simulink model "TurnLight1"  (R2020b)
settings: Solver=FixedStepDiscrete  StartTime=0.0  StopTime=10.0  FixedStep=0.01  RelTol=1e-3
values from neighbouring files (symbols this model uses):
  EBL_NO_REQ = 0    [TurnLightUserdata.m]
  EBL_REQ = 1    [TurnLightUserdata.m]
  HAZARDQR_OFF = 0    [TurnLightUserdata.m]
  HAZARDQR_ON = 1    [TurnLightUserdata.m]
  HAZARDRQ_OFF = 0    [TurnLightUserdata.m]
  HAZARDRQ_ON = 1    [TurnLightUserdata.m]
  HAZARDSW_OFF = 0    [TurnLightUserdata.m]
  HAZARDSW_ON = 1    [TurnLightUserdata.m]
  IGN_ACC = 1    [TurnLightUserdata.m]
  IGN_IGNST = 3    [TurnLightUserdata.m]
  IGN_OFF = 0    [TurnLightUserdata.m]
  IGN_ON = 2    [TurnLightUserdata.m]
  NO_CRASH = 0    [TurnLightUserdata.m]
  TLCC_ON = 1    [TurnLightUserdata.m]
  TLFB_OFF = 0    [TurnLightUserdata.m]
  TLFB_OPEN = 2    [TurnLightUserdata.m]
  TLFB_SHORT = 1    [TurnLightUserdata.m]
  TLSR_LEFT_ON = 1    [TurnLightUserdata.m]
  TLSR_OFF = 0    [TurnLightUserdata.m]
  TLSR_RIGHT_ON = 2    [TurnLightUserdata.m]
  TLSW_LEFT = 1    [TurnLightUserdata.m]
  TLSW_OFF = 0    [TurnLightUserdata.m]
  TLSW_RIGHT = 2    [TurnLightUserdata.m]
  TLSWMODE_FLASH0 = 0    [TurnLightUserdata.m]
  TLSWMODE_FLASH3 = 1    [TurnLightUserdata.m]
  TLSWMODE_FLASHLONG = 2    [TurnLightUserdata.m]
  VS_VALID = 1    [TurnLightUserdata.m]
undefined symbols (not defined in the file or in its folder): ComplexTurnLightONOFFType, ComplexTurnLightPositionType, TurnLightCtrlPara, TurnLightService_TurnLightControl_Operation
settings Model: Creator=Wangjianwen  LastModifiedBy=Wangjianwen
settings DataIOCC: SaveFormat=StructureWithTime
settings OptimizationCC: DefaultParameterBehavior=Inlined  EnhancedBackFolding=on  PassReuseOutputArgsAs=Individual arguments  ZeroExternalMemoryAtStartup=off  ZeroInternalMemoryAtStartup=off  OptimizeBlockOrder=speed  DifferentSizesBufferReuse=on  OptimizationCustomize=off  EfficientTunableParamExpr=on
settings DebuggingCC: ParameterTunabilityLossMsg=error  SFUnusedDataAndEventsDiag=none
settings HardwareCC: ProdLongLongMode=on
settings ModelReferenceCC: ModelReferenceNumInstancesAllowed=Single
settings SFSimCC: MATLABDynamicMemAlloc=off
settings RTWCC: Description=AUTOSAR  SystemTargetFile=autosar.tlc  GenCodeOnly=on  TemplateMakefile=ert_default_tmf
settings CodeAppCC: ForceParamTrailComments=on  IgnoreCustomStorageClasses=off  OperatorAnnotations=on  SimulinkDataObjDesc=on  SFDataObjDesc=on  InsertBlockDesc=on
settings STFCustomTargetCC: TargetLangStandard=C99 (ISO)  MultiwordLength=256  ParMdlRefBuildCompliant=on  CompOptLevelCompliant=on  ConcurrentExecutionCompliant=off  IncludeMdlTerminateFcn=off  CombineOutputUpdateFcns=on  SuppressErrorStatus=on  ERTCustomFileBanners=on  SupportNonFinite=off  SupportComplex=off  SupportContinuousTime=off  SupportNonInlinedSFcns=off  RemoveResetFunc=on  MATLABClassNameForMDSCustomization=Simulink.SoftwareTarget.ERTCustomization  CPPClassGenCompliant=off  AutosarCompliant=on  GRTInterface=off  UseToolchainInfoCompliant=on  LookupTableObjectStructAxisOrder=2,1,3,4,...  LUTObjectStructOrderEvenSpacing=Size,Table,Breakpoints  SystemTargetFile=autosar.tlc
settings ERTTargetCC: TargetLangStandard=C99 (ISO)  ConcurrentExecutionCompliant=off  IncludeMdlTerminateFcn=off  SuppressErrorStatus=on  SupportNonFinite=off  SupportComplex=off  ModelStepFunctionPrototypeControlCompliant=off  CPPClassGenCompliant=off  AutosarCompliant=on  LookupTableObjectStructAxisOrder=2,1,3,4,...  LUTObjectStructOrderEvenSpacing=Size,Table,Breakpoints  InlinedParameterPlacement=NonHierarchical  ERTCustomFileTemplate=example_file_process.tlc

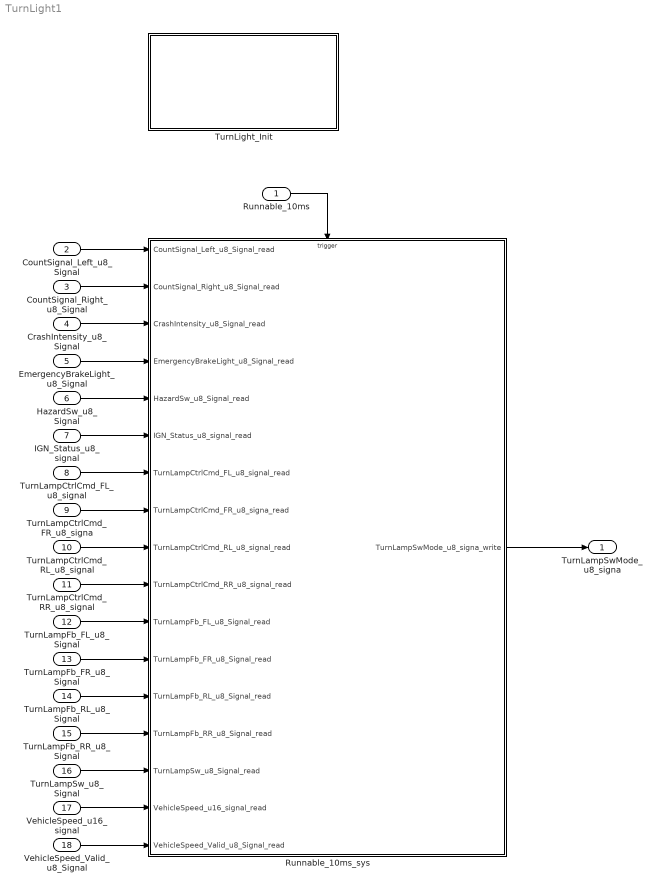
== system TurnLight1 ==
  Runnable_10ms : Inport  SampleTime=0.01  OutputFunctionCall=on
  CountSignal_Left_u8_Signal : Inport  Port=2  OutDataTypeStr=uint8  PortDimensions=1
  CountSignal_Right_u8_Signal : Inport  Port=3  OutDataTypeStr=uint8  PortDimensions=1
  CrashIntensity_u8_Signal : Inport  Port=4  OutDataTypeStr=uint8  PortDimensions=1
  EmergencyBrakeLight_u8_Signal : Inport  Port=5  OutDataTypeStr=uint8  PortDimensions=1
  HazardSw_u8_Signal : Inport  Port=6  OutDataTypeStr=uint8  PortDimensions=1
  IGN_Status_u8_signal : Inport  Port=7  OutDataTypeStr=uint8  PortDimensions=1
  TurnLampCtrlCmd_FL_u8_signal : Inport  Port=8  OutDataTypeStr=uint8  PortDimensions=1
  TurnLampCtrlCmd_FR_u8_signa : Inport  Port=9  OutDataTypeStr=uint8  PortDimensions=1
  TurnLampCtrlCmd_RL_u8_signal : Inport  Port=10  OutDataTypeStr=uint8  PortDimensions=1
  TurnLampCtrlCmd_RR_u8_signal : Inport  Port=11  OutDataTypeStr=uint64  PortDimensions=1
  TurnLampFb_FL_u8_Signal : Inport  Port=12  OutDataTypeStr=uint8  PortDimensions=1
  TurnLampFb_FR_u8_Signal : Inport  Port=13  OutDataTypeStr=uint8  PortDimensions=1
  TurnLampFb_RL_u8_Signal : Inport  Port=14  OutDataTypeStr=uint8  PortDimensions=1
  TurnLampFb_RR_u8_Signal : Inport  Port=15  OutDataTypeStr=uint8  PortDimensions=1
  TurnLampSw_u8_Signal : Inport  Port=16  OutDataTypeStr=uint8  PortDimensions=1
  VehicleSpeed_u16_signal : Inport  Port=17  OutDataTypeStr=uint16  PortDimensions=1
  VehicleSpeed_Valid_u8_Signal : Inport  Port=18  OutDataTypeStr=uint8  PortDimensions=1
  Runnable_10ms_sys : Subsystem
  TurnLight_Init : Subsystem
  TurnLampSwMode_u8_signa : Outport  OutDataTypeStr=uint8  PortDimensions=1
  wires:
  CountSignal_Left_u8_Signal/1 -> Runnable_10ms_sys/1(CountSignal_Left_u8_Signal_read)
  CountSignal_Right_u8_Signal/1 -> Runnable_10ms_sys/2(CountSignal_Right_u8_Signal_read)
  CrashIntensity_u8_Signal/1 -> Runnable_10ms_sys/3(CrashIntensity_u8_Signal_read)
  EmergencyBrakeLight_u8_Signal/1 -> Runnable_10ms_sys/4(EmergencyBrakeLight_u8_Signal_read)
  HazardSw_u8_Signal/1 -> Runnable_10ms_sys/5(HazardSw_u8_Signal_read)
  IGN_Status_u8_signal/1 -> Runnable_10ms_sys/6(IGN_Status_u8_signal_read)
  TurnLampCtrlCmd_FL_u8_signal/1 -> Runnable_10ms_sys/7(TurnLampCtrlCmd_FL_u8_signal_read)
  TurnLampCtrlCmd_FR_u8_signa/1 -> Runnable_10ms_sys/8(TurnLampCtrlCmd_FR_u8_signa_read)
  TurnLampCtrlCmd_RL_u8_signal/1 -> Runnable_10ms_sys/9(TurnLampCtrlCmd_RL_u8_signal_read)
  TurnLampCtrlCmd_RR_u8_signal/1 -> Runnable_10ms_sys/10(TurnLampCtrlCmd_RR_u8_signal_read)
  TurnLampFb_FL_u8_Signal/1 -> Runnable_10ms_sys/11(TurnLampFb_FL_u8_Signal_read)
  TurnLampFb_FR_u8_Signal/1 -> Runnable_10ms_sys/12(TurnLampFb_FR_u8_Signal_read)
  TurnLampFb_RL_u8_Signal/1 -> Runnable_10ms_sys/13(TurnLampFb_RL_u8_Signal_read)
  TurnLampFb_RR_u8_Signal/1 -> Runnable_10ms_sys/14(TurnLampFb_RR_u8_Signal_read)
  TurnLampSw_u8_Signal/1 -> Runnable_10ms_sys/15(TurnLampSw_u8_Signal_read)
  VehicleSpeed_u16_signal/1 -> Runnable_10ms_sys/16(VehicleSpeed_u16_signal_read)
  VehicleSpeed_Valid_u8_Signal/1 -> Runnable_10ms_sys/17(VehicleSpeed_Valid_u8_Signal_read)
  Runnable_10ms_sys/1(TurnLampSwMode_u8_signa_write) -> TurnLampSwMode_u8_signa/1
  Runnable_10ms/1 -> Runnable_10ms_sys/Trigger

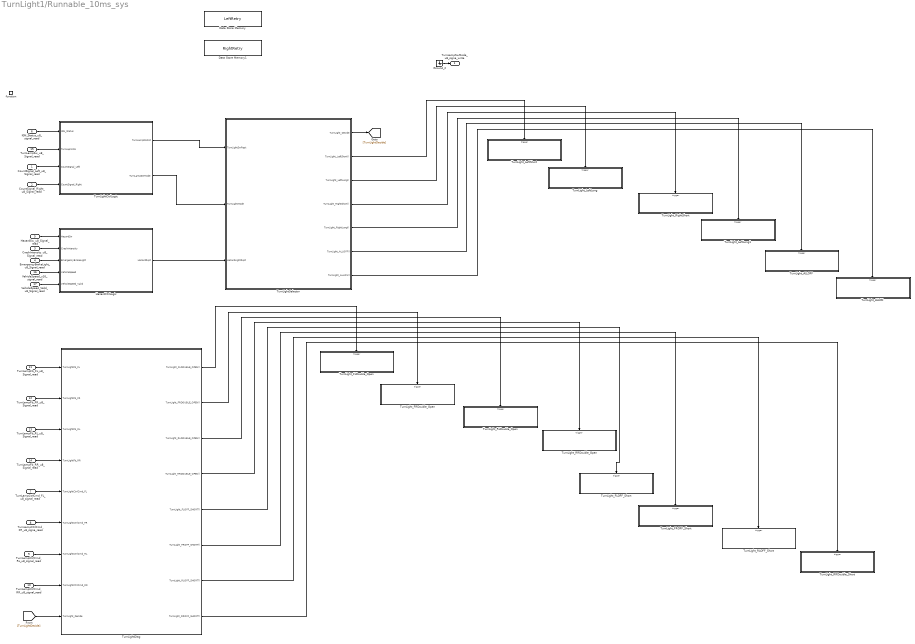
== system TurnLight1/Runnable_10ms_sys ==
  CountSignal_Left_u8_Signal_read : Inport
  CountSignal_Right_u8_Signal_read : Inport  Port=2
  CrashIntensity_u8_Signal_read : Inport  Port=3
  EmergencyBrakeLight_u8_Signal_read : Inport  Port=4
  HazardSw_u8_Signal_read : Inport  Port=5
  IGN_Status_u8_signal_read : Inport  Port=6
  TurnLampCtrlCmd_FL_u8_signal_read : Inport  Port=7
  TurnLampCtrlCmd_FR_u8_signa_read : Inport  Port=8
  TurnLampCtrlCmd_RL_u8_signal_read : Inport  Port=9
  TurnLampCtrlCmd_RR_u8_signal_read : Inport  Port=10
  TurnLampFb_FL_u8_Signal_read : Inport  Port=11
  TurnLampFb_FR_u8_Signal_read : Inport  Port=12
  TurnLampFb_RL_u8_Signal_read : Inport  Port=13
  TurnLampFb_RR_u8_Signal_read : Inport  Port=14
  TurnLampSw_u8_Signal_read : Inport  Port=15
  VehicleSpeed_u16_signal_read : Inport  Port=16
  VehicleSpeed_Valid_u8_Signal_read : Inport  Port=17
  function : TriggerPort  TriggerType=function-call  VariantControl=(inherit)  SampleTimeType=periodic  SampleTime=-1
  Data Store Memory : DataStoreMemory  DataStoreName=LeftRetry  ReadBeforeWriteMsg=warning  WriteAfterWriteMsg=warning  WriteAfterReadMsg=warning  ShowAdditionalParam=off  OutDataTypeStr=uint8
  Data Store Memory1 : DataStoreMemory  DataStoreName=RightRetry  ReadBeforeWriteMsg=warning  WriteAfterWriteMsg=warning  WriteAfterReadMsg=warning  ShowAdditionalParam=off  OutDataTypeStr=uint8
  Ground_2 : Ground
  HazardCtrlLogic : Stateflow chart  TreatAsAtomicUnit=on
  TurnLightCtrlLogic : Stateflow chart  TreatAsAtomicUnit=on
  TurnLightDiag : Stateflow chart  TreatAsAtomicUnit=on
  TurnLightSelector : Stateflow chart  TreatAsAtomicUnit=on
  TurnLight_ALLOFF : Subsystem
  TurnLight_ALLON : Subsystem
  TurnLight_FLDouble_Open : Subsystem
  TurnLight_FLOFF_Short : Subsystem
  TurnLight_FRDouble_Open : Subsystem
  TurnLight_FROFF_Short : Subsystem
  TurnLight_LeftLong : Subsystem
  TurnLight_LeftLong1 : Subsystem
  TurnLight_LeftShort : Subsystem
  TurnLight_RLDouble_Open : Subsystem
  TurnLight_RLOFF_Short : Subsystem
  TurnLight_RRDouble_Open : Subsystem
  TurnLight_RRDouble_Short : Subsystem
  TurnLight_RightShort : Subsystem
  TurnLampSwMode_u8_signa_write : Outport
      settings: EnsureOutportIsVirtual=on
  wires:
  CountSignal_Left_u8_Signal_read/1 -> TurnLightCtrlLogic/3(CountSignal_Left)
  CountSignal_Right_u8_Signal_read/1 -> TurnLightCtrlLogic/4(CountSignal_Right)
  CrashIntensity_u8_Signal_read/1 -> HazardCtrlLogic/2(CrashIntensity)
  EmergencyBrakeLight_u8_Signal_read/1 -> HazardCtrlLogic/3(EmergencyBrakeLight)
  HazardSw_u8_Signal_read/1 -> HazardCtrlLogic/1(HazardSw)
  TurnLampCtrlCmd_FL_u8_signal_read/1 -> TurnLightDiag/5(TurnLightCtrlCmd_FL)
  TurnLampCtrlCmd_FR_u8_signa_read/1 -> TurnLightDiag/6(TurnLightCtrlCmd_FR)
  TurnLampCtrlCmd_RL_u8_signal_read/1 -> TurnLightDiag/7(TurnLightCtrlCmd_RL)
  TurnLampCtrlCmd_RR_u8_signal_read/1 -> TurnLightDiag/8(TurnLightCtrlCmd_RR)
  TurnLampFb_FL_u8_Signal_read/1 -> TurnLightDiag/1(TurnLightFb_FL)
  TurnLampFb_FR_u8_Signal_read/1 -> TurnLightDiag/2(TurnLightFb_FR)
  TurnLampFb_RL_u8_Signal_read/1 -> TurnLightDiag/3(TurnLightFb_RL)
  TurnLampFb_RR_u8_Signal_read/1 -> TurnLightDiag/4(TurnLightFb_RR)
  TurnLampSw_u8_Signal_read/1 -> TurnLightCtrlLogic/2(TurnLapmSW)
  VehicleSpeed_u16_signal_read/1 -> HazardCtrlLogic/4(VehicleSpeed)
  VehicleSpeed_Valid_u8_Signal_read/1 -> HazardCtrlLogic/5(VehicleSpeed_Valid)
  Ground_2/1 -> TurnLampSwMode_u8_signa_write/1
  IGN_Status_u8_signal_read/1 -> TurnLightCtrlLogic/1(IGN_Status)
  TurnLightCtrlLogic/1(TurnLampSWRst) -> TurnLightSelector/1(TurnLightSwRqst)
  HazardCtrlLogic/1(HazardRqst) -> TurnLightSelector/3(HazardLightRqst)
  TurnLightCtrlLogic/2(TurnLampSWMode) -> TurnLightSelector/2(TurnLightMode)
  TurnLightSelector/2(TurnLight_LeftShort()) -> TurnLight_LeftShort/Trigger
  TurnLightSelector/3(TurnLight_LeftLong()) -> TurnLight_LeftLong/Trigger
  TurnLightSelector/4(TurnLight_RightShort()) -> TurnLight_RightShort/Trigger
  TurnLightSelector/5(TurnLight_RightLong()) -> TurnLight_LeftLong1/Trigger
  TurnLightSelector/6(TurnLight_ALLOFF()) -> TurnLight_ALLOFF/Trigger
  TurnLightSelector/7(TurnLight_ALLON()) -> TurnLight_ALLON/Trigger
  TurnLightSelector/1(TurnLight_Decide) -> [TurnLightDecide]
  [TurnLightDecide] -> TurnLightDiag/9(TurnLight_Decide)
  TurnLightDiag/1(TurnLight_FLDOUBLE_OPEN()) -> TurnLight_FLDouble_Open/Trigger
  TurnLightDiag/2(TurnLight_FRDOUBLE_OPEN()) -> TurnLight_FRDouble_Open/Trigger
  TurnLightDiag/3(TurnLight_RLDOUBLE_OPEN()) -> TurnLight_RLDouble_Open/Trigger
  TurnLightDiag/4(TurnLight_RRDOUBLE_OPEN()) -> TurnLight_RRDouble_Open/Trigger
  TurnLightDiag/5(TurnLight_FLOFF_SHORT()) -> TurnLight_FLOFF_Short/Trigger
  TurnLightDiag/6(TurnLight_FROFF_SHORT()) -> TurnLight_FROFF_Short/Trigger
  TurnLightDiag/7(TurnLight_RLOFF_SHORT()) -> TurnLight_RLOFF_Short/Trigger
  TurnLightDiag/8(TurnLight_RROFF_SHORT()) -> TurnLight_RRDouble_Short/Trigger

== system TurnLight1/TurnLight_Init ==
  Event Listener : EventListener  EventName=reset

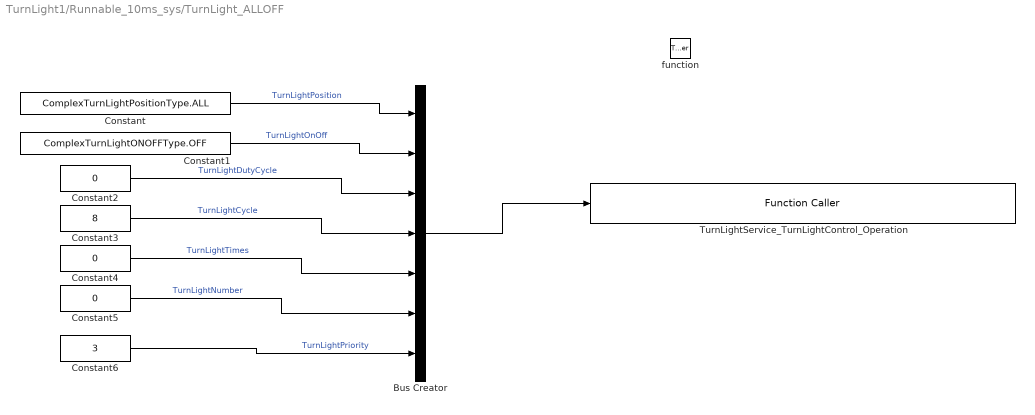
== system TurnLight1/Runnable_10ms_sys/TurnLight_ALLOFF ==
  function : TriggerPort  TriggerType=function-call  VariantControl=Variant
  Bus Creator : BusCreator  Inputs=7  OutDataTypeStr=Bus: TurnLightService  NonVirtualBus=on
  Constant : Constant  Value=ComplexTurnLightPositionType.ALL  OutDataTypeStr=Enum: ComplexTurnLightPositionType
  Constant1 : Constant  Value=ComplexTurnLightONOFFType.OFF  OutDataTypeStr=Enum: ComplexTurnLightONOFFType
  Constant2 : Constant  Value=0  OutDataTypeStr=uint8
  Constant3 : Constant  Value=8  OutDataTypeStr=uint8
  Constant4 : Constant  Value=0  OutDataTypeStr=uint8
  Constant5 : Constant  Value=0  OutDataTypeStr=uint8
  Constant6 : Constant  Value=3  OutDataTypeStr=uint8
  TurnLightService_TurnLightControl_Operation : FunctionCaller  FunctionPrototype=TurnLightService_TurnLightControl_Operation(TurnLightCtrlPara)  InputArgumentSpecifications=P_TurnLightService
  wires:
  Constant6/1 -> Bus Creator/7  "TurnLightPriority"
  Constant5/1 -> Bus Creator/6  "TurnLightNumber"
  Constant4/1 -> Bus Creator/5  "TurnLightTimes"
  Constant3/1 -> Bus Creator/4  "TurnLightCycle"
  Constant2/1 -> Bus Creator/3  "TurnLightDutyCycle"
  Constant1/1 -> Bus Creator/2  "TurnLightOnOff"
  Constant/1 -> Bus Creator/1  "TurnLightPosition"
  Bus Creator/1 -> TurnLightService_TurnLightControl_Operation/1

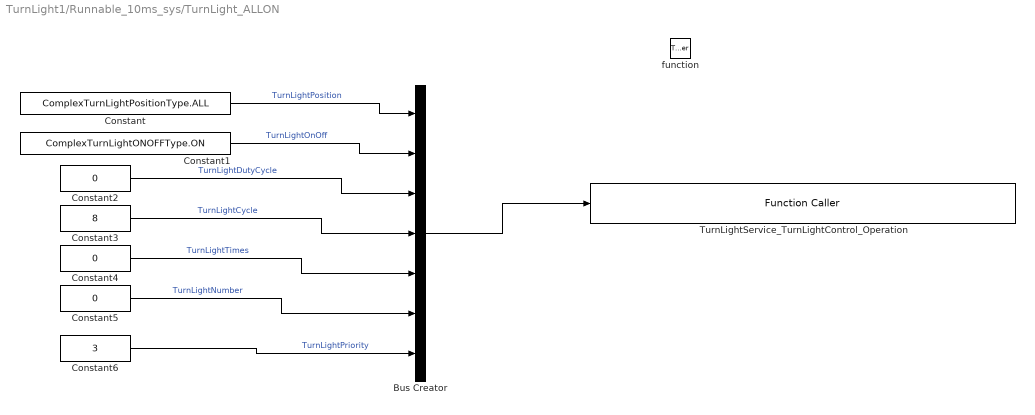
== system TurnLight1/Runnable_10ms_sys/TurnLight_ALLON ==
  function : TriggerPort  TriggerType=function-call  VariantControl=Variant
  Bus Creator : BusCreator  Inputs=7  OutDataTypeStr=Bus: TurnLightService  NonVirtualBus=on
  Constant : Constant  Value=ComplexTurnLightPositionType.ALL  OutDataTypeStr=Enum: ComplexTurnLightPositionType
  Constant1 : Constant  Value=ComplexTurnLightONOFFType.ON  OutDataTypeStr=Enum: ComplexTurnLightONOFFType
  Constant2 : Constant  Value=0  OutDataTypeStr=uint8
  Constant3 : Constant  Value=8  OutDataTypeStr=uint8
  Constant4 : Constant  Value=0  OutDataTypeStr=uint8
  Constant5 : Constant  Value=0  OutDataTypeStr=uint8
  Constant6 : Constant  Value=3  OutDataTypeStr=uint8
  TurnLightService_TurnLightControl_Operation : FunctionCaller  FunctionPrototype=TurnLightService_TurnLightControl_Operation(TurnLightCtrlPara)  InputArgumentSpecifications=P_TurnLightService
  wires:
  Bus Creator/1 -> TurnLightService_TurnLightControl_Operation/1
  Constant/1 -> Bus Creator/1  "TurnLightPosition"
  Constant1/1 -> Bus Creator/2  "TurnLightOnOff"
  Constant2/1 -> Bus Creator/3  "TurnLightDutyCycle"
  Constant3/1 -> Bus Creator/4  "TurnLightCycle"
  Constant4/1 -> Bus Creator/5  "TurnLightTimes"
  Constant5/1 -> Bus Creator/6  "TurnLightNumber"
  Constant6/1 -> Bus Creator/7  "TurnLightPriority"

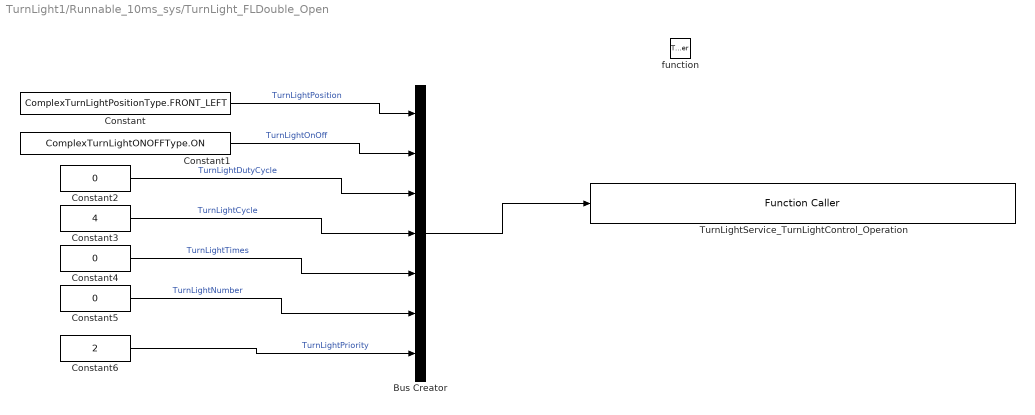
== system TurnLight1/Runnable_10ms_sys/TurnLight_FLDouble_Open ==
  function : TriggerPort  TriggerType=function-call  VariantControl=Variant
  Bus Creator : BusCreator  Inputs=7  OutDataTypeStr=Bus: TurnLightService  NonVirtualBus=on
  Constant : Constant  Value=ComplexTurnLightPositionType.FRONT_LEFT  OutDataTypeStr=Enum: ComplexTurnLightPositionType
  Constant1 : Constant  Value=ComplexTurnLightONOFFType.ON  OutDataTypeStr=Enum: ComplexTurnLightONOFFType
  Constant2 : Constant  Value=0  OutDataTypeStr=uint8
  Constant3 : Constant  Value=4  OutDataTypeStr=uint8
  Constant4 : Constant  Value=0  OutDataTypeStr=uint8
  Constant5 : Constant  Value=0  OutDataTypeStr=uint8
  Constant6 : Constant  Value=2  OutDataTypeStr=uint8
  TurnLightService_TurnLightControl_Operation : FunctionCaller  FunctionPrototype=TurnLightService_TurnLightControl_Operation(TurnLightCtrlPara)  InputArgumentSpecifications=P_TurnLightService
  wires:
  Bus Creator/1 -> TurnLightService_TurnLightControl_Operation/1
  Constant/1 -> Bus Creator/1  "TurnLightPosition"
  Constant1/1 -> Bus Creator/2  "TurnLightOnOff"
  Constant2/1 -> Bus Creator/3  "TurnLightDutyCycle"
  Constant3/1 -> Bus Creator/4  "TurnLightCycle"
  Constant4/1 -> Bus Creator/5  "TurnLightTimes"
  Constant5/1 -> Bus Creator/6  "TurnLightNumber"
  Constant6/1 -> Bus Creator/7  "TurnLightPriority"

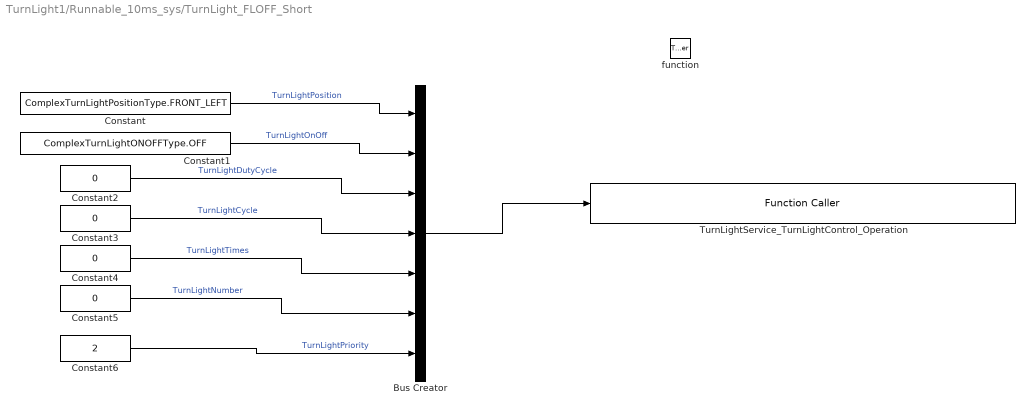
== system TurnLight1/Runnable_10ms_sys/TurnLight_FLOFF_Short ==
  function : TriggerPort  TriggerType=function-call  VariantControl=Variant
  Bus Creator : BusCreator  Inputs=7  OutDataTypeStr=Bus: TurnLightService  NonVirtualBus=on
  Constant : Constant  Value=ComplexTurnLightPositionType.FRONT_LEFT  OutDataTypeStr=Enum: ComplexTurnLightPositionType
  Constant1 : Constant  Value=ComplexTurnLightONOFFType.OFF  OutDataTypeStr=Enum: ComplexTurnLightONOFFType
  Constant{2..5} (4 alike) : Constant  Value=0  OutDataTypeStr=uint8
  Constant6 : Constant  Value=2  OutDataTypeStr=uint8
  TurnLightService_TurnLightControl_Operation : FunctionCaller  FunctionPrototype=TurnLightService_TurnLightControl_Operation(TurnLightCtrlPara)  InputArgumentSpecifications=P_TurnLightService
  wires:
  Constant6/1 -> Bus Creator/7  "TurnLightPriority"
  Constant5/1 -> Bus Creator/6  "TurnLightNumber"
  Constant4/1 -> Bus Creator/5  "TurnLightTimes"
  Constant3/1 -> Bus Creator/4  "TurnLightCycle"
  Constant2/1 -> Bus Creator/3  "TurnLightDutyCycle"
  Constant1/1 -> Bus Creator/2  "TurnLightOnOff"
  Constant/1 -> Bus Creator/1  "TurnLightPosition"
  Bus Creator/1 -> TurnLightService_TurnLightControl_Operation/1

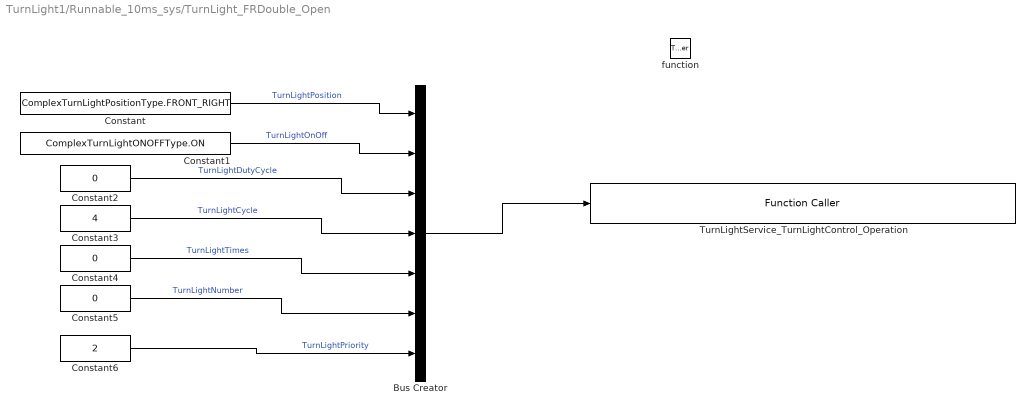
== system TurnLight1/Runnable_10ms_sys/TurnLight_FRDouble_Open ==
  function : TriggerPort  TriggerType=function-call  VariantControl=Variant
  Bus Creator : BusCreator  Inputs=7  OutDataTypeStr=Bus: TurnLightService  NonVirtualBus=on
  Constant : Constant  Value=ComplexTurnLightPositionType.FRONT_RIGHT  OutDataTypeStr=Enum: ComplexTurnLightPositionType
  Constant1 : Constant  Value=ComplexTurnLightONOFFType.ON  OutDataTypeStr=Enum: ComplexTurnLightONOFFType
  Constant2 : Constant  Value=0  OutDataTypeStr=uint8
  Constant3 : Constant  Value=4  OutDataTypeStr=uint8
  Constant4 : Constant  Value=0  OutDataTypeStr=uint8
  Constant5 : Constant  Value=0  OutDataTypeStr=uint8
  Constant6 : Constant  Value=2  OutDataTypeStr=uint8
  TurnLightService_TurnLightControl_Operation : FunctionCaller  FunctionPrototype=TurnLightService_TurnLightControl_Operation(TurnLightCtrlPara)  InputArgumentSpecifications=P_TurnLightService
  wires:
  Constant6/1 -> Bus Creator/7  "TurnLightPriority"
  Constant5/1 -> Bus Creator/6  "TurnLightNumber"
  Constant4/1 -> Bus Creator/5  "TurnLightTimes"
  Constant3/1 -> Bus Creator/4  "TurnLightCycle"
  Constant2/1 -> Bus Creator/3  "TurnLightDutyCycle"
  Constant1/1 -> Bus Creator/2  "TurnLightOnOff"
  Constant/1 -> Bus Creator/1  "TurnLightPosition"
  Bus Creator/1 -> TurnLightService_TurnLightControl_Operation/1

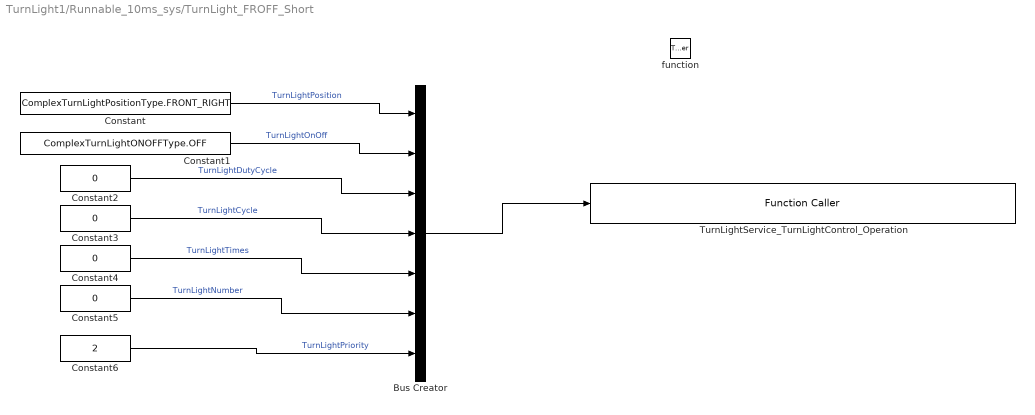
== system TurnLight1/Runnable_10ms_sys/TurnLight_FROFF_Short ==
  function : TriggerPort  TriggerType=function-call  VariantControl=Variant
  Bus Creator : BusCreator  Inputs=7  OutDataTypeStr=Bus: TurnLightService  NonVirtualBus=on
  Constant : Constant  Value=ComplexTurnLightPositionType.FRONT_RIGHT  OutDataTypeStr=Enum: ComplexTurnLightPositionType
  Constant1 : Constant  Value=ComplexTurnLightONOFFType.OFF  OutDataTypeStr=Enum: ComplexTurnLightONOFFType
  Constant{2..5} (4 alike) : Constant  Value=0  OutDataTypeStr=uint8
  Constant6 : Constant  Value=2  OutDataTypeStr=uint8
  TurnLightService_TurnLightControl_Operation : FunctionCaller  FunctionPrototype=TurnLightService_TurnLightControl_Operation(TurnLightCtrlPara)  InputArgumentSpecifications=P_TurnLightService
  wires:
  Bus Creator/1 -> TurnLightService_TurnLightControl_Operation/1
  Constant/1 -> Bus Creator/1  "TurnLightPosition"
  Constant1/1 -> Bus Creator/2  "TurnLightOnOff"
  Constant2/1 -> Bus Creator/3  "TurnLightDutyCycle"
  Constant3/1 -> Bus Creator/4  "TurnLightCycle"
  Constant4/1 -> Bus Creator/5  "TurnLightTimes"
  Constant5/1 -> Bus Creator/6  "TurnLightNumber"
  Constant6/1 -> Bus Creator/7  "TurnLightPriority"

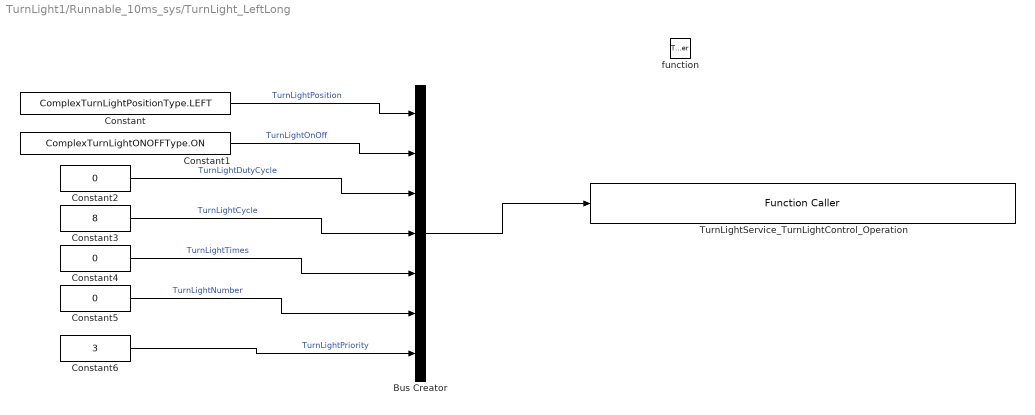
== system TurnLight1/Runnable_10ms_sys/TurnLight_LeftLong ==
  function : TriggerPort  TriggerType=function-call  VariantControl=Variant
  Bus Creator : BusCreator  Inputs=7  OutDataTypeStr=Bus: TurnLightService  NonVirtualBus=on
  Constant : Constant  Value=ComplexTurnLightPositionType.LEFT  OutDataTypeStr=Enum: ComplexTurnLightPositionType
  Constant1 : Constant  Value=ComplexTurnLightONOFFType.ON  OutDataTypeStr=Enum: ComplexTurnLightONOFFType
  Constant2 : Constant  Value=0  OutDataTypeStr=uint8
  Constant3 : Constant  Value=8  OutDataTypeStr=uint8
  Constant4 : Constant  Value=0  OutDataTypeStr=uint8
  Constant5 : Constant  Value=0  OutDataTypeStr=uint8
  Constant6 : Constant  Value=3  OutDataTypeStr=uint8
  TurnLightService_TurnLightControl_Operation : FunctionCaller  FunctionPrototype=TurnLightService_TurnLightControl_Operation(TurnLightCtrlPara)  InputArgumentSpecifications=P_TurnLightService
  wires:
  Constant6/1 -> Bus Creator/7  "TurnLightPriority"
  Constant5/1 -> Bus Creator/6  "TurnLightNumber"
  Constant4/1 -> Bus Creator/5  "TurnLightTimes"
  Constant3/1 -> Bus Creator/4  "TurnLightCycle"
  Constant2/1 -> Bus Creator/3  "TurnLightDutyCycle"
  Constant1/1 -> Bus Creator/2  "TurnLightOnOff"
  Constant/1 -> Bus Creator/1  "TurnLightPosition"
  Bus Creator/1 -> TurnLightService_TurnLightControl_Operation/1

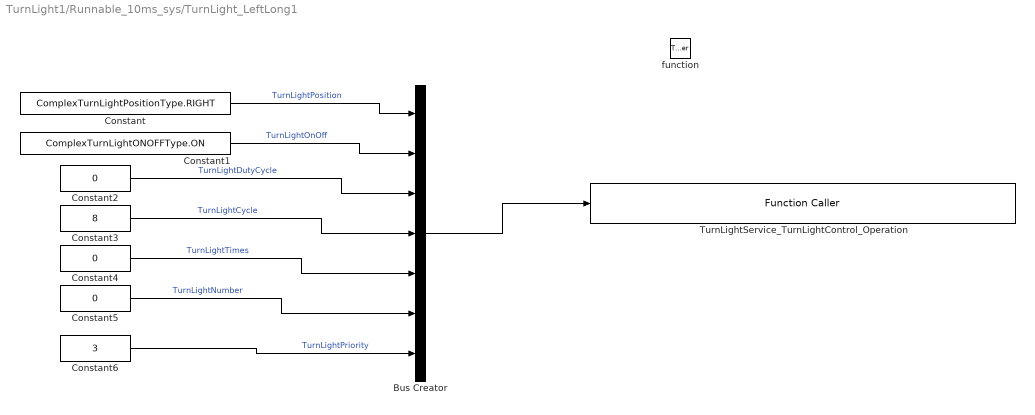
== system TurnLight1/Runnable_10ms_sys/TurnLight_LeftLong1 ==
  function : TriggerPort  TriggerType=function-call  VariantControl=Variant
  Bus Creator : BusCreator  Inputs=7  OutDataTypeStr=Bus: TurnLightService  NonVirtualBus=on
  Constant : Constant  Value=ComplexTurnLightPositionType.RIGHT  OutDataTypeStr=Enum: ComplexTurnLightPositionType
  Constant1 : Constant  Value=ComplexTurnLightONOFFType.ON  OutDataTypeStr=Enum: ComplexTurnLightONOFFType
  Constant2 : Constant  Value=0  OutDataTypeStr=uint8
  Constant3 : Constant  Value=8  OutDataTypeStr=uint8
  Constant4 : Constant  Value=0  OutDataTypeStr=uint8
  Constant5 : Constant  Value=0  OutDataTypeStr=uint8
  Constant6 : Constant  Value=3  OutDataTypeStr=uint8
  TurnLightService_TurnLightControl_Operation : FunctionCaller  FunctionPrototype=TurnLightService_TurnLightControl_Operation(TurnLightCtrlPara)  InputArgumentSpecifications=P_TurnLightService
  wires:
  Bus Creator/1 -> TurnLightService_TurnLightControl_Operation/1
  Constant/1 -> Bus Creator/1  "TurnLightPosition"
  Constant1/1 -> Bus Creator/2  "TurnLightOnOff"
  Constant2/1 -> Bus Creator/3  "TurnLightDutyCycle"
  Constant3/1 -> Bus Creator/4  "TurnLightCycle"
  Constant4/1 -> Bus Creator/5  "TurnLightTimes"
  Constant5/1 -> Bus Creator/6  "TurnLightNumber"
  Constant6/1 -> Bus Creator/7  "TurnLightPriority"

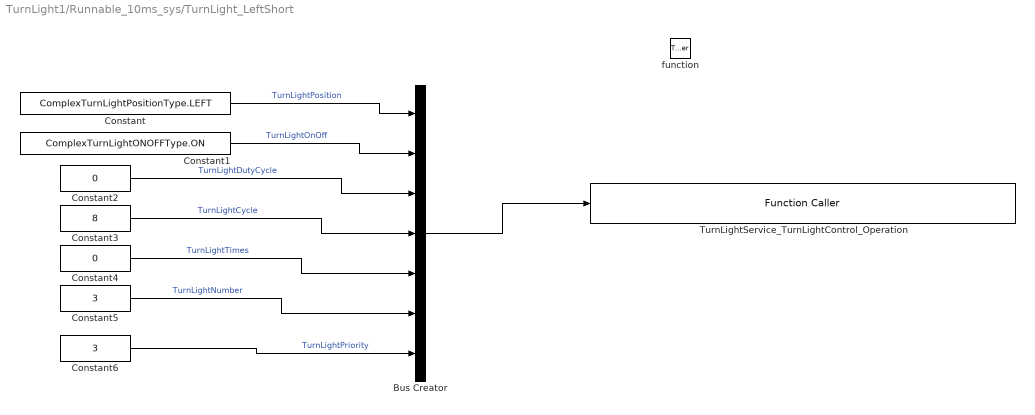
== system TurnLight1/Runnable_10ms_sys/TurnLight_LeftShort ==
  function : TriggerPort  TriggerType=function-call  VariantControl=Variant
  Bus Creator : BusCreator  Inputs=7  OutDataTypeStr=Bus: TurnLightService  NonVirtualBus=on
  Constant : Constant  Value=ComplexTurnLightPositionType.LEFT  OutDataTypeStr=Enum: ComplexTurnLightPositionType
  Constant1 : Constant  Value=ComplexTurnLightONOFFType.ON  OutDataTypeStr=Enum: ComplexTurnLightONOFFType
  Constant2 : Constant  Value=0  OutDataTypeStr=uint8
  Constant3 : Constant  Value=8  OutDataTypeStr=uint8
  Constant4 : Constant  Value=0  OutDataTypeStr=uint8
  Constant5 : Constant  Value=3  OutDataTypeStr=uint8
  Constant6 : Constant  Value=3  OutDataTypeStr=uint8
  TurnLightService_TurnLightControl_Operation : FunctionCaller  FunctionPrototype=TurnLightService_TurnLightControl_Operation(TurnLightCtrlPara)  InputArgumentSpecifications=P_TurnLightService
  wires:
  Bus Creator/1 -> TurnLightService_TurnLightControl_Operation/1
  Constant/1 -> Bus Creator/1  "TurnLightPosition"
  Constant1/1 -> Bus Creator/2  "TurnLightOnOff"
  Constant2/1 -> Bus Creator/3  "TurnLightDutyCycle"
  Constant3/1 -> Bus Creator/4  "TurnLightCycle"
  Constant4/1 -> Bus Creator/5  "TurnLightTimes"
  Constant5/1 -> Bus Creator/6  "TurnLightNumber"
  Constant6/1 -> Bus Creator/7  "TurnLightPriority"

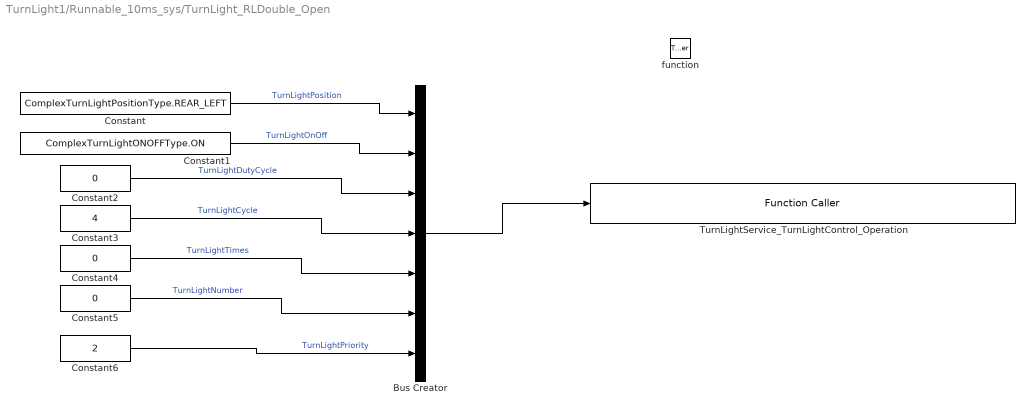
== system TurnLight1/Runnable_10ms_sys/TurnLight_RLDouble_Open ==
  function : TriggerPort  TriggerType=function-call  VariantControl=Variant
  Bus Creator : BusCreator  Inputs=7  OutDataTypeStr=Bus: TurnLightService  NonVirtualBus=on
  Constant : Constant  Value=ComplexTurnLightPositionType.REAR_LEFT  OutDataTypeStr=Enum: ComplexTurnLightPositionType
  Constant1 : Constant  Value=ComplexTurnLightONOFFType.ON  OutDataTypeStr=Enum: ComplexTurnLightONOFFType
  Constant2 : Constant  Value=0  OutDataTypeStr=uint8
  Constant3 : Constant  Value=4  OutDataTypeStr=uint8
  Constant4 : Constant  Value=0  OutDataTypeStr=uint8
  Constant5 : Constant  Value=0  OutDataTypeStr=uint8
  Constant6 : Constant  Value=2  OutDataTypeStr=uint8
  TurnLightService_TurnLightControl_Operation : FunctionCaller  FunctionPrototype=TurnLightService_TurnLightControl_Operation(TurnLightCtrlPara)  InputArgumentSpecifications=P_TurnLightService
  wires:
  Bus Creator/1 -> TurnLightService_TurnLightControl_Operation/1
  Constant/1 -> Bus Creator/1  "TurnLightPosition"
  Constant1/1 -> Bus Creator/2  "TurnLightOnOff"
  Constant2/1 -> Bus Creator/3  "TurnLightDutyCycle"
  Constant3/1 -> Bus Creator/4  "TurnLightCycle"
  Constant4/1 -> Bus Creator/5  "TurnLightTimes"
  Constant5/1 -> Bus Creator/6  "TurnLightNumber"
  Constant6/1 -> Bus Creator/7  "TurnLightPriority"

== system TurnLight1/Runnable_10ms_sys/TurnLight_RLOFF_Short ==
  function : TriggerPort  TriggerType=function-call  VariantControl=Variant
  Bus Creator : BusCreator  Inputs=7  OutDataTypeStr=Bus: TurnLightService  NonVirtualBus=on
  Constant : Constant  Value=ComplexTurnLightPositionType.REAR_LEFT  OutDataTypeStr=Enum: ComplexTurnLightPositionType
  Constant1 : Constant  Value=ComplexTurnLightONOFFType.OFF  OutDataTypeStr=Enum: ComplexTurnLightONOFFType
  Constant{2..5} (4 alike) : Constant  Value=0  OutDataTypeStr=uint8
  Constant6 : Constant  Value=2  OutDataTypeStr=uint8
  TurnLightService_TurnLightControl_Operation : FunctionCaller  FunctionPrototype=TurnLightService_TurnLightControl_Operation(TurnLightCtrlPara)  InputArgumentSpecifications=P_TurnLightService
  wires:
  Constant6/1 -> Bus Creator/7  "TurnLightPriority"
  Constant5/1 -> Bus Creator/6  "TurnLightNumber"
  Constant4/1 -> Bus Creator/5  "TurnLightTimes"
  Constant3/1 -> Bus Creator/4  "TurnLightCycle"
  Constant2/1 -> Bus Creator/3  "TurnLightDutyCycle"
  Constant1/1 -> Bus Creator/2  "TurnLightOnOff"
  Constant/1 -> Bus Creator/1  "TurnLightPosition"
  Bus Creator/1 -> TurnLightService_TurnLightControl_Operation/1

== system TurnLight1/Runnable_10ms_sys/TurnLight_RRDouble_Open ==
  function : TriggerPort  TriggerType=function-call  VariantControl=Variant
  Bus Creator : BusCreator  Inputs=7  OutDataTypeStr=Bus: TurnLightService  NonVirtualBus=on
  Constant : Constant  Value=ComplexTurnLightPositionType.REAR_RIGHT  OutDataTypeStr=Enum: ComplexTurnLightPositionType
  Constant1 : Constant  Value=ComplexTurnLightONOFFType.ON  OutDataTypeStr=Enum: ComplexTurnLightONOFFType
  Constant2 : Constant  Value=0  OutDataTypeStr=uint8
  Constant3 : Constant  Value=4  OutDataTypeStr=uint8
  Constant4 : Constant  Value=0  OutDataTypeStr=uint8
  Constant5 : Constant  Value=0  OutDataTypeStr=uint8
  Constant6 : Constant  Value=2  OutDataTypeStr=uint8
  TurnLightService_TurnLightControl_Operation : FunctionCaller  FunctionPrototype=TurnLightService_TurnLightControl_Operation(TurnLightCtrlPara)  InputArgumentSpecifications=P_TurnLightService
  wires:
  Constant6/1 -> Bus Creator/7  "TurnLightPriority"
  Constant5/1 -> Bus Creator/6  "TurnLightNumber"
  Constant4/1 -> Bus Creator/5  "TurnLightTimes"
  Constant3/1 -> Bus Creator/4  "TurnLightCycle"
  Constant2/1 -> Bus Creator/3  "TurnLightDutyCycle"
  Constant1/1 -> Bus Creator/2  "TurnLightOnOff"
  Constant/1 -> Bus Creator/1  "TurnLightPosition"
  Bus Creator/1 -> TurnLightService_TurnLightControl_Operation/1

== system TurnLight1/Runnable_10ms_sys/TurnLight_RRDouble_Short ==
  function : TriggerPort  TriggerType=function-call  VariantControl=Variant
  Bus Creator : BusCreator  Inputs=7  OutDataTypeStr=Bus: TurnLightService  NonVirtualBus=on
  Constant : Constant  Value=ComplexTurnLightPositionType.REAR_RIGHT  OutDataTypeStr=Enum: ComplexTurnLightPositionType
  Constant1 : Constant  Value=ComplexTurnLightONOFFType.OFF  OutDataTypeStr=Enum: ComplexTurnLightONOFFType
  Constant{2..5} (4 alike) : Constant  Value=0  OutDataTypeStr=uint8
  Constant6 : Constant  Value=2  OutDataTypeStr=uint8
  TurnLightService_TurnLightControl_Operation : FunctionCaller  FunctionPrototype=TurnLightService_TurnLightControl_Operation(TurnLightCtrlPara)  InputArgumentSpecifications=P_TurnLightService
  wires:
  Bus Creator/1 -> TurnLightService_TurnLightControl_Operation/1
  Constant/1 -> Bus Creator/1  "TurnLightPosition"
  Constant1/1 -> Bus Creator/2  "TurnLightOnOff"
  Constant2/1 -> Bus Creator/3  "TurnLightDutyCycle"
  Constant3/1 -> Bus Creator/4  "TurnLightCycle"
  Constant4/1 -> Bus Creator/5  "TurnLightTimes"
  Constant5/1 -> Bus Creator/6  "TurnLightNumber"
  Constant6/1 -> Bus Creator/7  "TurnLightPriority"

== system TurnLight1/Runnable_10ms_sys/TurnLight_RightShort ==
  function : TriggerPort  TriggerType=function-call  VariantControl=Variant
  Bus Creator : BusCreator  Inputs=7  OutDataTypeStr=Bus: TurnLightService  NonVirtualBus=on
  Constant : Constant  Value=ComplexTurnLightPositionType.RIGHT  OutDataTypeStr=Enum: ComplexTurnLightPositionType
  Constant1 : Constant  Value=ComplexTurnLightONOFFType.ON  OutDataTypeStr=Enum: ComplexTurnLightONOFFType
  Constant2 : Constant  Value=0  OutDataTypeStr=uint8
  Constant3 : Constant  Value=8  OutDataTypeStr=uint8
  Constant4 : Constant  Value=0  OutDataTypeStr=uint8
  Constant5 : Constant  Value=3  OutDataTypeStr=uint8
  Constant6 : Constant  Value=3  OutDataTypeStr=uint8
  TurnLightService_TurnLightControl_Operation : FunctionCaller  FunctionPrototype=TurnLightService_TurnLightControl_Operation(TurnLightCtrlPara)  InputArgumentSpecifications=P_TurnLightService
  wires:
  Constant6/1 -> Bus Creator/7  "TurnLightPriority"
  Constant5/1 -> Bus Creator/6  "TurnLightNumber"
  Constant4/1 -> Bus Creator/5  "TurnLightTimes"
  Constant3/1 -> Bus Creator/4  "TurnLightCycle"
  Constant2/1 -> Bus Creator/3  "TurnLightDutyCycle"
  Constant1/1 -> Bus Creator/2  "TurnLightOnOff"
  Constant/1 -> Bus Creator/1  "TurnLightPosition"
  Bus Creator/1 -> TurnLightService_TurnLightControl_Operation/1

== stateflow chart TurnLight1/Runnable_10ms_sys/HazardCtrlLogic ==
  state OFF
    en:
    HazardRqst = HAZARDRQ_OFF;
  state ON_Crash
    en:
    HazardRqst = HAZARDRQ_ON;
  state On_EmergencyBrake
    en:
    HazardRqst = HAZARDRQ_ON;
  state ON_SW
    en:
    HazardRqst = HAZARDRQ_ON;
  (default) -> OFF
  OFF -> ON_Crash [order 1] : [hasChangedFrom(CrashIntensity,NO_CRASH)]
  ON_Crash -> OFF [order 1] : [CrashIntensity~=NO_CRASH &&after(500,tick)&&hasChangedTo(HazardSw,HAZARDSW_ON)]
  ON_Crash -> OFF [order 2] : [CrashIntensity~=NO_CRASH && after(90000,tick)]
  OFF -> On_EmergencyBrake [order 2] : [hasChangedTo(EmergencyBrakeLight,EBL_REQ)]
  On_EmergencyBrake -> OFF [order 1] : [EmergencyBrakeLight == EBL_REQ&&hasChangedTo(HazardSw,HAZARDSW_ON)]
  On_EmergencyBrake -> OFF [order 2] : [EmergencyBrakeLight ==EBL_REQ&&VehicleSpeed>15&&VehicleSpeed_Valid ==VS_VALID]
  OFF -> ON_SW [order 3] : [hasChangedTo(HazardSw,HAZARDSW_ON)]
  ON_SW -> OFF : [hasChangedTo(HazardSw,HAZARDSW_ON)]
  data: HazardSw input; CrashIntensity input; EmergencyBrakeLight input; VehicleSpeed input; VehicleSpeed_Valid input; HazardRqst output uint8 =0; NO_CRASH parameter uint8; EBL_NO_REQ parameter uint8; EBL_REQ parameter uint8; VS_VALID parameter uint8; HAZARDSW_OFF parameter uint8; HAZARDSW_ON parameter uint8; HAZARDQR_OFF parameter uint8; HAZARDQR_ON parameter uint8; HAZARDRQ_OFF parameter; HAZARDRQ_ON parameter

== stateflow chart TurnLight1/Runnable_10ms_sys/TurnLightSelector ==
  state DecideLeftLongOrShort [function]
    (default) -> (junction 94) : /* 决策闪烁模式 */
    (junction 94) -> (junction 95) [order 1] : [TurnLightMode == TLSWMODE_FLASH3]
    (junction 94) -> (junction 96) [order 2] : {TurnLight_LeftLong; TurnLight_Decide = TurnLightDecideStType.LEFTLONG;}
    (junction 95) -> (junction 97) : {TurnLight_LeftShort; TurnLight_Decide = TurnLightDecideStType.LEFTSHORT;}
    (junction 97) -> (junction 96)
    (junction 96) -> (junction 98)
  state DecideRightLongOrShort [function]
    (default) -> (junction 104) : /* 决策闪烁模式 */
    (junction 104) -> (junction 106) [order 1] : [TurnLightMode == TLSWMODE_FLASH3]
    (junction 104) -> (junction 108) [order 2] : {TurnLight_RightLong; TurnLight_Decide = TurnLightDecideStType.RIGHTLONG;}
    (junction 106) -> (junction 107) : {TurnLight_RightShort; TurnLight_Decide = TurnLightDecideStType.RIGHTSHORT;}
    (junction 107) -> (junction 108)
    (junction 108) -> (junction 110)
  state LEFTON
    en:
    LeftRetry = 0;
    DecideLeftLongOrShort();
  state ALLOFF
    en:
    TurnLight_ALLOFF
    TurnLight_Decide = TurnLightDecideStType.ALLOFF;
  state RIGHTON
    en:
    RightRetry = 0;
    DecideRightLongOrShort();
  state ALLON
    en:
    TurnLight_ALLON
    TurnLight_Decide = TurnLightDecideStType.ALLON;
  LEFTON -> LEFTON [order 4] : [LeftRetry ==1]
  (default) -> ALLOFF
  LEFTON -> (junction 21) [order 1] : [TurnLightSwRqst == TLSR_LEFT_ON && hasChangedTo(HazardLightRqst,HAZARDRQ_ON)]
  (junction 21) -> (junction 23)
  ALLOFF -> LEFTON [order 1] : [TurnLightSwRqst == TLSR_LEFT_ON]
  LEFTON -> (junction 26) [order 2] : [HazardLightRqst == HAZARDRQ_ON && hasChangedFrom(TurnLightSwRqst,TLSR_LEFT_ON)]
  (junction 26) -> (junction 28)
  LEFTON -> ALLOFF [order 3] : [TurnLightSwRqst ==TLSR_OFF]
  (junction 31) -> LEFTON
  (junction 36) -> (junction 31)
  (junction 32) -> LEFTON
  (junction 40) -> (junction 32)
  RIGHTON -> RIGHTON [order 4] : [RightRetry ==1]
  RIGHTON -> (junction 51) [order 1] : [TurnLightSwRqst == TLSR_RIGHT_ON && hasChangedTo(HazardLightRqst,HAZARDRQ_ON)]
  (junction 51) -> (junction 45)
  ALLOFF -> RIGHTON [order 2] : [TurnLightSwRqst == TLSR_RIGHT_ON]
  RIGHTON -> (junction 56) [order 2] : [HazardLightRqst == HAZARDRQ_ON && hasChangedFrom(TurnLightSwRqst,TLSR_RIGHT_ON)]
  (junction 56) -> (junction 60)
  (junction 59) -> RIGHTON
  (junction 48) -> (junction 59)
  RIGHTON -> ALLOFF [order 3] : [TurnLightSwRqst == TLSR_OFF]
  (junction 62) -> RIGHTON
  (junction 55) -> (junction 62)
  ALLOFF -> ALLON [order 3] : [HazardLightRqst == HAZARDRQ_ON]
  ALLON -> (junction 55) [order 3] : [TurnLightSwRqst == TLSR_RIGHT_ON && hasChangedTo(HazardLightRqst,HAZARDQR_OFF)]
  ALLON -> (junction 48) [order 1] : [HazardLightRqst == HAZARDQR_ON && hasChangedTo(TurnLightSwRqst,TLSR_RIGHT_ON)]
  (junction 60) -> ALLON
  (junction 45) -> ALLON
  ALLON -> ALLOFF [order 5] : [HazardLightRqst == HAZARDRQ_OFF]
  ALLON -> (junction 40) [order 4] : [TurnLightSwRqst == TLSR_LEFT_ON && hasChangedTo(HazardLightRqst,HAZARDQR_OFF)]
  ALLON -> (junction 36) [order 2] : [HazardLightRqst == HAZARDQR_ON && hasChangedTo(TurnLightSwRqst,TLSR_LEFT_ON)]
  (junction 28) -> ALLON
  (junction 23) -> ALLON
  data: TurnLightSwRqst input; TurnLightMode input; HazardLightRqst input; TLSR_OFF parameter uint8; TLSR_LEFT_ON parameter uint8; TLSR_RIGHT_ON parameter uint8; HAZARDQR_ON parameter uint8; HAZARDQR_OFF parameter uint8; TLSWMODE_FLASH3 parameter uint8; TLSWMODE_FLASHLONG parameter uint8; TurnLight_Decide output uint8; LeftRetry data_store_memory; RightRetry data_store_memory; HAZARDRQ_OFF parameter; HAZARDRQ_ON parameter
  events: TurnLight_LeftShort output FUNCTION_CALL_EVENT; TurnLight_LeftLong output FUNCTION_CALL_EVENT; TurnLight_RightShort output FUNCTION_CALL_EVENT; TurnLight_RightLong output FUNCTION_CALL_EVENT; TurnLight_ALLOFF output FUNCTION_CALL_EVENT; TurnLight_ALLON output FUNCTION_CALL_EVENT

== stateflow chart TurnLight1/Runnable_10ms_sys/TurnLightCtrlLogic ==
  state IDLE
    en:
    TurnLampSWMode = 0;
    TurnLampSWRst = 0;
    TurnLapmCount = 0;
  state LEFT
    state Check1
      en,du:TurnLapmCount = TurnLapmCount+1;
    state Check2
      en:
      TurnLampSWRst = TLSR_LEFT_ON;
      du:
      TurnLapmCount = TurnLapmCount+1;
    state ShortFlash
      en:
      TurnLampSWMode = TLSWMODE_FLASH3;
    state LongFlash
      en:
      TurnLampSWMode = TLSWMODE_FLASHLONG;
    LEFT.Check1 -> LEFT.Check2 [order 2] : [TurnLapmCount >10]
    LEFT.Check2 -> LEFT.ShortFlash [order 1] : [TurnLapmCount <=70&&TurnLapmSW == TLSW_OFF ]
    LEFT.Check2 -> LEFT.LongFlash [order 2] : [TurnLapmCount >70&&TurnLapmSW == TLSW_LEFT]
  state RIGHT
    state Check1
      en,du:TurnLapmCount = TurnLapmCount+1;
    state Check2
      en:
      TurnLampSWRst = TLSR_RIGHT_ON;
      du:
      TurnLapmCount = TurnLapmCount+1;
    state ShortFlash
      en:
      TurnLampSWMode = TLSWMODE_FLASH3;
    state LongFlash
      en:
      TurnLampSWMode = TLSWMODE_FLASHLONG;
    RIGHT.Check1 -> RIGHT.Check2 [order 2] : [TurnLapmCount >10]
    RIGHT.Check2 -> RIGHT.ShortFlash [order 1] : [TurnLapmCount <=70&&TurnLapmSW == TLSW_OFF ]
    RIGHT.Check2 -> RIGHT.LongFlash [order 2] : [TurnLapmCount >70&&TurnLapmSW == TLSW_RIGHT]
  (default) -> IDLE
  IDLE -> LEFT.Check1 [order 1] : [(IGN_Status== IGN_ON || IGN_Status ==IGN_IGNST)&&...
      | TurnLapmSW == TLSW_LEFT]
  LEFT.Check1 -> IDLE [order 1] : [TurnLapmSW ~= TLSW_LEFT]
  LEFT.ShortFlash -> IDLE : [CountSignal_Left == 3]
  LEFT.LongFlash -> IDLE : [TurnLapmSW == TLSW_OFF &&...
      | (IGN_Status == IGN_OFF|| IGN_Status == IGN_ACC )]
  IDLE -> RIGHT.Check1 [order 2] : [(IGN_Status== IGN_ON || IGN_Status ==IGN_IGNST)&&...
      | TurnLapmSW == TLSW_RIGHT]
  RIGHT.Check1 -> IDLE [order 1] : [TurnLapmSW ~= TLSW_RIGHT]
  RIGHT.ShortFlash -> IDLE : [CountSignal_Left == 3]
  RIGHT.LongFlash -> IDLE : [TurnLapmSW == TLSW_OFF &&...
      | (IGN_Status == IGN_OFF|| IGN_Status == IGN_ACC )]
  data: IGN_Status input; TurnLapmSW input; CountSignal_Left input; CountSignal_Right input; TurnLampSWRst output uint8 =0; TurnLampSWMode output uint8 =0; TurnLapmCount local uint8; IGN_OFF parameter uint8; IGN_ACC parameter uint8; IGN_ON parameter uint8; IGN_IGNST parameter uint8; TLSW_OFF parameter uint8; TLSW_LEFT parameter uint8; TLSW_RIGHT parameter uint8; TLSR_OFF parameter uint8; TLSR_LEFT_ON parameter uint8; TLSR_RIGHT_ON parameter uint8; TLSWMODE_FLASH0 parameter uint8; TLSWMODE_FLASH3 parameter uint8; TLSWMODE_FLASHLONG parameter uint8

== stateflow chart TurnLight1/Runnable_10ms_sys/TurnLightDiag ==
  state FLDIAG [parallel]
    settings: executionOrder=1
    state SHORT
      en:
      FL_DIAGSt = DiagStType.SHORT;
      TurnLight_FLOFF_SHORT
    state IDLE
      en:
      FL_DIAGSt = DiagStType.NORMAL;
    state OPEN
      en:
      FL_DIAGSt = DiagStType.OPEN;
      TurnLight_FLDOUBLE_OPEN
    (default) -> FLDIAG.IDLE
    FLDIAG.IDLE -> FLDIAG.SHORT [order 1] : [TurnLightFb_FL == TLFB_SHORT...
        | &&TurnLightCtrlCmd_FL ==TLCC_ON]
    FLDIAG.SHORT -> FLDIAG.IDLE : [TurnLight_Decide == TurnLightDecideStType.ALLOFF]
    FLDIAG.IDLE -> FLDIAG.OPEN [order 2] : [TurnLightFb_FL == TLFB_OPEN...
        | &&TurnLightCtrlCmd_FL ==TLCC_ON]
    FLDIAG.OPEN -> FLDIAG.IDLE : [TurnLightFb_FL == TLFB_OFF]{LeftRetry =1}
  state FRDIAG [parallel]
    settings: executionOrder=2
    state SHORT
      en:
      FR_DIAGSt = DiagStType.SHORT;
      TurnLight_FROFF_SHORT
    state IDLE
      en:
      FL_DIAGSt = DiagStType.NORMAL;
    state OPEN
      en:
      FR_DIAGSt = DiagStType.OPEN;
      TurnLight_FRDOUBLE_OPEN
    (default) -> FRDIAG.IDLE
    FRDIAG.IDLE -> FRDIAG.SHORT [order 1] : [TurnLightFb_FR == TLFB_SHORT...
        | &&TurnLightCtrlCmd_FR ==TLCC_ON]
    FRDIAG.SHORT -> FRDIAG.IDLE : [TurnLight_Decide == TurnLightDecideStType.ALLOFF]
    FRDIAG.IDLE -> FRDIAG.OPEN [order 2] : [TurnLightFb_FR == TLFB_OPEN...
        | &&TurnLightCtrlCmd_FR ==TLCC_ON]
    FRDIAG.OPEN -> FRDIAG.IDLE : [TurnLightFb_FR == TLFB_OFF]{RightRetry =1}
  state RLDIAG [parallel]
    settings: executionOrder=3
    state SHORT
      en:
      RL_DIAGSt = DiagStType.SHORT;
      TurnLight_RLOFF_SHORT
    state IDLE
      en:
      FL_DIAGSt = DiagStType.NORMAL;
    state OPEN
      en:
      RL_DIAGSt = DiagStType.OPEN;
      TurnLight_RLDOUBLE_OPEN
    (default) -> RLDIAG.IDLE
    RLDIAG.IDLE -> RLDIAG.SHORT [order 1] : [TurnLightFb_RL == TLFB_SHORT...
        | &&TurnLightCtrlCmd_RL ==TLCC_ON]
    RLDIAG.SHORT -> RLDIAG.IDLE : [TurnLight_Decide == TurnLightDecideStType.ALLOFF]
    RLDIAG.IDLE -> RLDIAG.OPEN [order 2] : [TurnLightFb_RL == TLFB_OPEN...
        | &&TurnLightCtrlCmd_FL ==TLCC_ON]
    RLDIAG.OPEN -> RLDIAG.IDLE : [TurnLightFb_RL == TLFB_OFF]{LeftRetry =1}
  state RRDIAG [parallel]
    settings: executionOrder=4
    state SHORT
      en:
      FL_DIAGSt = DiagStType.SHORT;
      TurnLight_RROFF_SHORT
    state IDLE
      en:
      FL_DIAGSt = DiagStType.NORMAL;
    state OPEN
      en:
      FL_DIAGSt = DiagStType.OPEN;
      TurnLight_RRDOUBLE_OPEN
    (default) -> RRDIAG.IDLE
    RRDIAG.IDLE -> RRDIAG.SHORT [order 1] : [TurnLightFb_FL == TLFB_SHORT...
        | &&TurnLightCtrlCmd_FL ==TLCC_ON]
    RRDIAG.SHORT -> RRDIAG.IDLE : [TurnLight_Decide == TurnLightDecideStType.ALLOFF]
    RRDIAG.IDLE -> RRDIAG.OPEN [order 2] : [TurnLightFb_FL == TLFB_OPEN...
        | &&TurnLightCtrlCmd_FL ==TLCC_ON]
    RRDIAG.OPEN -> RRDIAG.IDLE : [TurnLightFb_FL == TLFB_OFF]{RightRetry =1}
  data: TurnLightFb_FL input; TurnLightFb_FR input; TurnLightFb_RL input; TurnLightFb_RR input; TurnLightCtrlCmd_FL input; TurnLightCtrlCmd_FR input; TurnLightCtrlCmd_RL input; TurnLightCtrlCmd_RR input; FL_DIAGSt local uint8; FR_DIAGSt local uint8; RL_DIAGSt local uint8; RR_DIAGSt local uint8; TurnLight_Decide input uint8; LeftRetry data_store_memory; RightRetry data_store_memory; TLCC_ON parameter; TLFB_OFF parameter; TLFB_OPEN parameter; TLFB_SHORT parameter
  events: TurnLight_FLDOUBLE_OPEN output FUNCTION_CALL_EVENT; TurnLight_FRDOUBLE_OPEN output FUNCTION_CALL_EVENT; TurnLight_RLDOUBLE_OPEN output FUNCTION_CALL_EVENT; TurnLight_RRDOUBLE_OPEN output FUNCTION_CALL_EVENT; TurnLight_FLOFF_SHORT output FUNCTION_CALL_EVENT; TurnLight_FROFF_SHORT output FUNCTION_CALL_EVENT; TurnLight_RLOFF_SHORT output FUNCTION_CALL_EVENT; TurnLight_RROFF_SHORT output FUNCTION_CALL_EVENT
